simulink model "Model_LQR_Real"  (R2025a)
settings: Solver=ode4  StartTime=0.0  StopTime=inf  FixedStep=0.00001  RelTol=1e-3
InitFcn:
  | addpath('functions');
model workspace: external: MATLAB File D:\OneDrive - University of Bristol\2025-2026\grp-major_project - General\LQR\furuta-inverted-pendulum-LQR\init_LQR.m (data not in the file)
values from neighbouring files (symbols this model uses):
  alpha = 0.8    [init_LQR.m]
  c_omega = (N_gear^2 * Kt * Ke) / R_motor    (= 0.00492477886361)    [init_LQR.m]
  c_V = (N_gear * Kt) / R_motor    (= 0.0277237642805)    [init_LQR.m]
  fric_1 = [f_v_1, f_c_1, k_fc_1]    [furuta_single_inverted_pendulum_nonlive_copy.m]    (also in init_LQR.m)
  fric_arm = [f_v_arm, f_c_arm, k_fc_arm]    [furuta_single_inverted_pendulum_nonlive_copy.m]    (also in init_LQR.m)
  I_1 = in2(:,4)    [furuta_single_A_B_matrices.m]    (also in furuta_single_state_derivative.m = in4(:,4); init_LQR.m = 0.00011)
  I_arm = in2(:,2)    [furuta_single_A_B_matrices.m]    (also in furuta_single_state_derivative.m = in4(:,2); init_LQR.m = 0.000739)
  init_S = [0; 0; 0.26; 0]    [init_LQR.m]
  K_voltage = lqr(A_new, B_new, Q, R)    [init_LQR.m]
  L_1 = 0.14    [init_LQR.m]    (also in playback_animation_single.m = out.plotData.L_1.Data(1))
  L_arm = in2(:,1)    [furuta_single_A_B_matrices.m]    (also in furuta_single_state_derivative.m = in4(:,1); init_LQR.m = 0.1475; playback_animation_single.m = out.plotData.L_arm.Data(1))
  lcom_1 = in2(:,3)    [furuta_single_A_B_matrices.m]    (also in furuta_single_state_derivative.m = in4(:,3); init_LQR.m = 0.051; playback_animation_single.m = out.plotData.lcom_1.Data(1))
  m_1 = in2(:,5)    [furuta_single_A_B_matrices.m]    (also in furuta_single_state_derivative.m = in4(:,5); init_LQR.m = 0.054)
libraries: simulink x4
settings Model: PacingRate=0.071000  Creator=Esther  LastModifiedBy=Hankin

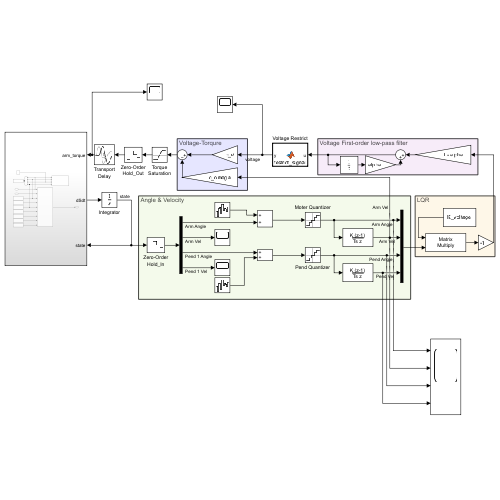
[thumbnail: Simulink's stored preview of the top-level diagram]
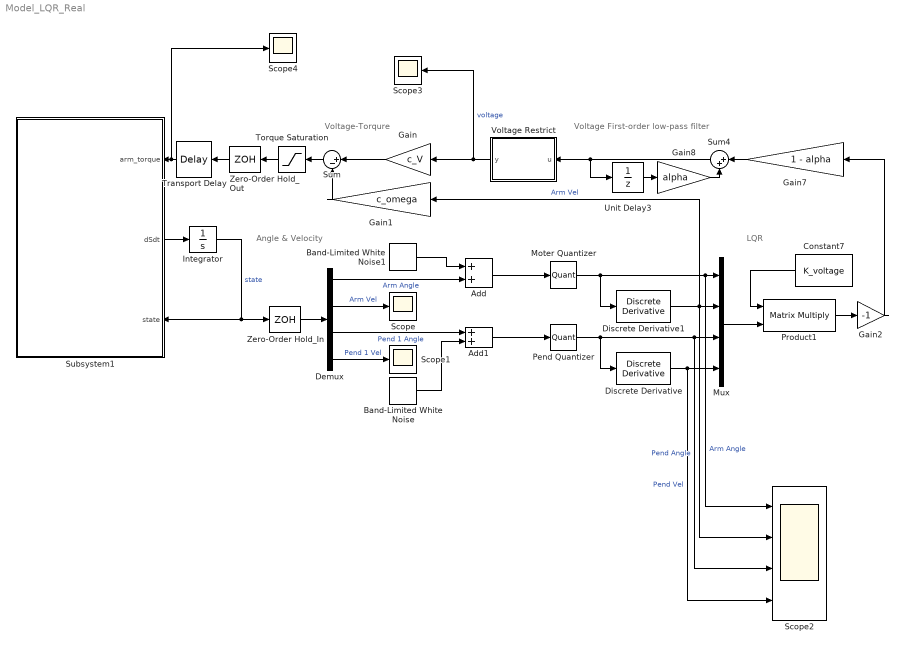
== system Model_LQR_Real ==
  note: Voltage First-order low-pass filter
  note: LQR
  note: Angle & Velocity
  note: Voltage-Torqure
  Add : Sum
  Add1 : Sum
  Band-Limited White Noise : simulink/Sources/Band-Limited White Noise  Cov=[1e-9]  Ts=0.001  seed=[23341]  VectorParams1D=off
  Band-Limited White Noise1 : simulink/Sources/Band-Limited White Noise  Cov=[1e-9]  Ts=0.001  seed=[23341]  VectorParams1D=off
  Constant7 : Constant  Value=K_voltage  VectorParams1D=off
  Demux : Demux
  Discrete Derivative : simulink/Discrete/Discrete Derivative  gainval=1.0  ICPrevScaledInput=0.0  OutMin=[]  OutMax=[]  OutDataType=fixdt(1, 16)  OutScaling=2^-10  DoSatur=off
  Discrete Derivative1 : simulink/Discrete/Discrete Derivative  gainval=1.0  ICPrevScaledInput=0.0  OutMin=[]  OutMax=[]  OutDataType=fixdt(1, 16)  OutScaling=2^-10  DoSatur=off
  Gain : Gain  Gain=c_V
  Gain1 : Gain  Gain=c_omega
  Gain2 : Gain  Gain=-1
  Gain7 : Gain  Gain=1 - alpha
  Gain8 : Gain  Gain=alpha
  Integrator : Integrator  InitialCondition=init_S
  Moter Quantizer : Quantizer  QuantizationInterval=2*pi/408  LinearizeAsGain=off
  Mux : Mux
  Pend Quantizer : Quantizer  QuantizationInterval=2*pi/8000  LinearizeAsGain=off
  Product1 : Product  Multiplication=Matrix(*)
  Scope{,1,3..4} (4 alike) : Scope
      Scope settings: ActiveDisplayYMinimum=-1  ActiveDisplayYMaximum=1
      Scope3 settings: ActiveDisplayYMinimum=-2.5340953879528954  ActiveDisplayYMaximum=1.3219005521989886  DataLoggingVariableName=ScopeData3
      Scope4 settings: ActiveDisplayYMinimum=-0.1007987796316209  ActiveDisplayYMaximum=0.1089776421812912  DataLoggingVariableName=ScopeData4
  Scope2 : Scope  NumInputPorts=4
      settings: ActiveDisplayString=4  ActiveDisplayYMinimum=-9.17903023911575  ActiveDisplayYMaximum=5.2758684361494685  DataLoggingVariableName=ScopeData2
  Subsystem1 : Subsystem
      settings: PortSchema="{\"entries\":[{\"content\":{\"sides\":[{\"content\":{},\"type\":\"ConnectorPlacement.EquallySpacedRectSide\",\"uuid\":\"5a98f0b0-99f4-4816-b10a-c8507da40489\"},{\"content\":{\"connectorIds\":[\"In1\",\"Out1\",\"In2\"],\"side\":\"RIGHT\"},\"type\":\"ConnectorPlacement.EquallySpacedRectSide\",\"uuid\":\"8494f5bf-2264-4508-933b-fad8bf72c107\"},{\"content\":{\"side\":\"TOP\"},\"type\":\"ConnectorPlacement.EquallySpacedRectSide\",\"uuid\":\"2309ac97-33c2-43e6-877e-a0383f3dff2f\"}]},\"type\":\"ConnectorPlacement.EquallySpacedConnector\",\"uuid\":\"880f2894-8eee-450d-b899-a591cd1fba41\"}],\"packageUris\":[\"http://schema.mathworks.com/mf0/Connector/R2020b\"],\"version\":\"1.0\"}"
  Sum : Sum  Inputs=|+-
  Sum4 : Sum  Inputs=|++
  Torque Saturation : Saturate  UpperLimit=0.088  LowerLimit=-0.088  LinearizeAsGain=off
  Transport Delay : TransportDelay  DelayTime=0.0003
  Unit Delay3 : UnitDelay  InputProcessing=Columns as channels (frame based)  SampleTime=-1  HasFrameUpgradeWarning=on
  Voltage Restrict : MATLAB Function  TreatAsAtomicUnit=on
  Zero-Order Hold_In : ZeroOrderHold  SampleTime=0.001
  Zero-Order Hold_Out : ZeroOrderHold  SampleTime=0.001
  wires:
  Integrator/1 -> Zero-Order Hold_In/1, Subsystem1/2(state)  "state"
  Sum/1 -> Torque Saturation/1
  Product1/1 -> Gain2/1
  Zero-Order Hold_In/1 -> Demux/1
  Constant7/1 -> Product1/1
  Demux/2 -> Scope/1  "Arm Vel"
  Demux/4 -> Scope1/1  "Pend 1 Vel"
  Voltage Restrict/1(y) -> Gain/1, Scope3/1  "voltage"
  Subsystem1/1(dSdt) -> Integrator/1
  Mux/1 -> Product1/2
  Moter Quantizer/1 -> Discrete Derivative1/1, Scope2/1, Mux/1  "Arm Angle"
  Discrete Derivative1/1 -> Gain1/1, Scope2/2, Mux/2  "Arm Vel"
  Discrete Derivative/1 -> Scope2/4, Mux/4  "Pend Vel"
  Pend Quantizer/1 -> Discrete Derivative/1, Scope2/3, Mux/3  "Pend Angle"
  Gain/1 -> Sum/1
  Gain1/1 -> Sum/2
  Zero-Order Hold_Out/1 -> Transport Delay/1
  Add/1 -> Moter Quantizer/1
  Demux/1 -> Add/2  "Arm Angle"
  Add1/1 -> Pend Quantizer/1
  Demux/3 -> Add1/1  "Pend 1 Angle"
  Band-Limited White Noise/1 -> Add1/2
  Band-Limited White Noise1/1 -> Add/1
  Transport Delay/1 -> Subsystem1/1(arm_torque), Scope4/1
  Gain7/1 -> Sum4/1
  Unit Delay3/1 -> Gain8/1
  Gain8/1 -> Sum4/2
  Gain2/1 -> Gain7/1
  Torque Saturation/1 -> Zero-Order Hold_Out/1
  Sum4/1 -> Voltage Restrict/1(u), Unit Delay3/1

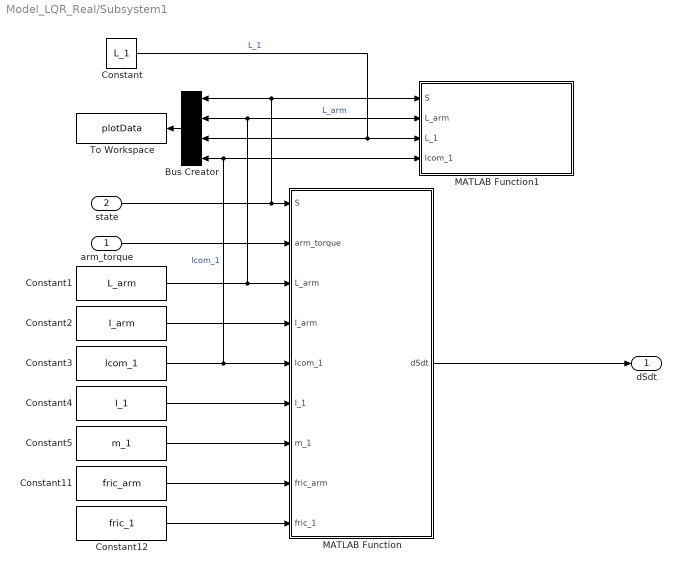
== system Model_LQR_Real/Subsystem1 ==
  arm_torque : Inport
  state : Inport  Port=2
  Bus Creator : BusCreator  Inputs=4
  Constant : Constant  Value=L_1
  Constant1 : Constant  Value=L_arm
  Constant11 : Constant  Value=fric_arm  VectorParams1D=off
  Constant12 : Constant  Value=fric_1  VectorParams1D=off
  Constant2 : Constant  Value=I_arm
  Constant3 : Constant  Value=lcom_1
  Constant4 : Constant  Value=I_1
  Constant5 : Constant  Value=m_1
  MATLAB Function : MATLAB Function  TreatAsAtomicUnit=on
  MATLAB Function1 : MATLAB Function  TreatAsAtomicUnit=on
  To Workspace : ToWorkspace  VariableName=plotData  SaveFormat=Timeseries  SampleTime=-1
  dSdt : Outport
  wires:
  Constant4/1 -> MATLAB Function/6(I_1)
  Bus Creator/1 -> To Workspace/1
  Constant1/1 -> MATLAB Function1/2(L_arm), Bus Creator/2, MATLAB Function/3(L_arm)  "L_arm"
  Constant3/1 -> Bus Creator/4, MATLAB Function1/4(lcom_1), MATLAB Function/5(lcom_1)  "lcom_1"
  Constant5/1 -> MATLAB Function/7(m_1)
  Constant2/1 -> MATLAB Function/4(I_arm)
  Constant/1 -> MATLAB Function1/3(L_1), Bus Creator/3  "L_1"
  state/1 -> Bus Creator/1, MATLAB Function1/1(S), MATLAB Function/1(S)
  MATLAB Function/1(dSdt) -> dSdt/1
  arm_torque/1 -> MATLAB Function/2(arm_torque)
  Constant11/1 -> MATLAB Function/8(fric_arm)
  Constant12/1 -> MATLAB Function/9(fric_1)

== matlab function Model_LQR_Real/Subsystem1/MATLAB Function1 ==
  settings: updateMethod=DISCRETE
  data: S input; L_arm input; L_1 input; lcom_1 input
function animation(S, L_arm, L_1, lcom_1)
    update_ratio = 100;
    realtime_animation_single(S, L_arm, L_1, lcom_1, update_ratio);
end

== matlab function Model_LQR_Real/Subsystem1/MATLAB Function ==
  data: S input size=4; dSdt output size=4; arm_torque input size=1; L_arm input size=1; I_arm input size=1; lcom_1 input size=1; I_1 input size=1; m_1 input size=1; fric_arm input; fric_1 input
function dSdt = get_dSdt(S, arm_torque, L_arm, I_arm, lcom_1, I_1, m_1, fric_arm, fric_1)
    t = 0;
    g = 9.81;
    phys_param = [L_arm, I_arm, lcom_1, I_1, m_1, g];
    dSdt = furuta_single_state_derivative(t, S, arm_torque, phys_param, fric_arm, fric_1);
end

== matlab function Model_LQR_Real/Voltage Restrict ==
  data: u input; y output
function y = restrict_signal(u)
      % 限制最大值和最小值
      if u > 12
          y = 12;
      elseif u < -12
          y = -12;
      % 限制中心剔除区间 (-0.6, 0.6)
      % 将非负微小信号钳位至正区间下限
      elseif u >= 0 && u < 0.6
          y = 0;
      % 将负微小信号钳位至负区间上限
      elseif u < 0 && u > -0.6
          y = 0;
      % 信号在正常区间 [-12, -0.6] 或 [0.6, 12] 内，保持原值
      else
          y = u;
      end
  end
